simulink model "s_b8a4x128f"  (R2016b)
settings: Solver=VariableStepDiscrete  StartTime=0.0  StopTime=1  RelTol=1e-3
undefined symbols (not defined in the file): fft_stages, n_bits_ants, n_bits_xengs
libraries: xbsIndex_r4 x21069, casper_library_misc x164, casper_library_scopes x9, xbsReplacements_r4 x9, casper_library_delays x8, xps_library x3
(part 27 of 186)

== system s_b8a4x128f/sys1/bf_pack_out1 ==
  note: ensure sync_in
      | aligns with data
      | for storage
      | in FIFO
  note: rst turns off
      | as first data item
      | becomes available
      | at fifo
  note: insert dead time (based on clock rates and packet size) before transmission to guarantee this
      | packet will not overflow the fifo. Note that this assumes destination fifo at least as large as the packet
  note: if in reset report
      | end of file
      | immediately
  note: if there is an overflow, flush
      | all buffers and reset logic. Then
      | hold in reset till next sync
  note: increment heap offset
      | as packets leave
  note: keep space for
      | two timestamps/syncs
  note: change timestamp/sync
      | as last packet of
      | heap leaves
  note: capture timestamp on
      | first data item
      | of heap
  rst : Inport
  synci : Inport  Port=2
  di : Inport  Port=3
  eni : Inport  Port=4
  timei : Inport  Port=5
  start : Inport  Port=6
  id : Inport  Port=7
  Assert1 : xbsIndex_r4/Assert  assert_type=on  type_source=Explicitly  gui_display_data_type=Fixed-point  arith_type=Unsigned  n_bits=group_size_bits  bin_pt=0  preci_type=Single  exp_width=8  frac_width=24  assert_rate=off  rate_source=Explicitly  period=1  output_port=on  block_type=assert
      settings: block_version=11.4
  Assert{2,4,6,10} (4 alike) : xbsIndex_r4/Assert  assert_type=on  type_source=Explicitly  gui_display_data_type=Fixed-point  arith_type=Boolean  n_bits=1  bin_pt=0  preci_type=Single  exp_width=8  frac_width=24  assert_rate=off  rate_source=Explicitly  period=1  output_port=on  block_type=assert
      settings: block_version=11.4
  Assert5 : xbsIndex_r4/Assert  assert_type=on  type_source=Explicitly  gui_display_data_type=Fixed-point  arith_type=Unsigned  n_bits=spead_lsw  bin_pt=0  preci_type=Single  exp_width=8  frac_width=24  assert_rate=off  rate_source=Explicitly  period=1  output_port=on  block_type=assert
      settings: block_version=11.4
  Assert7 : xbsIndex_r4/Assert  assert_type=on  type_source=Explicitly  gui_display_data_type=Fixed-point  arith_type=Unsigned  n_bits=8*2^bit_width_in  bin_pt=0  preci_type=Single  exp_width=8  frac_width=24  assert_rate=off  rate_source=Explicitly  period=1  output_port=on  block_type=assert
      settings: block_version=11.4
  Concat{,1..3} (4 alike) : xbsIndex_r4/Concat  num_inputs=2  dbl_ovrd=off  block_type=concat
  Constant : xbsIndex_r4/Constant  const=0  gui_display_data_type=Fixed-point  arith_type=Signed (2's comp)  n_bits=heap_bits  bin_pt=0  preci_type=Single  exp_width=8  frac_width=24  explicit_period=off  period=1  equ=P=C  opselect=C  inp2=PCIN>>17  opr=+  inp1=P  carry=CIN  dbl_ovrd=off  block_type=constant
      settings: block_version=11.4
  Constant1 : xbsIndex_r4/Constant  const=0  gui_display_data_type=Fixed-point  arith_type=Unsigned  n_bits=48  bin_pt=0  preci_type=Single  exp_width=8  frac_width=24  explicit_period=on  period=1  equ=P=C  opselect=C  inp2=PCIN>>17  opr=+  inp1=P  carry=CIN  dbl_ovrd=off  block_type=constant
  Constant2 : xbsIndex_r4/Constant  const=2^(packet_bits-bit_width_out)  gui_display_data_type=Fixed-point  arith_type=Unsigned  n_bits=48  bin_pt=0  preci_type=Single  exp_width=8  frac_width=24  explicit_period=on  period=1  equ=P=C  opselect=C  inp2=PCIN>>17  opr=+  inp1=P  carry=CIN  dbl_ovrd=off  block_type=constant
  Constant3 : xbsIndex_r4/Constant  const=0  gui_display_data_type=Fixed-point  arith_type=Unsigned  n_bits=packet_bits  bin_pt=0  preci_type=Single  exp_width=8  frac_width=24  explicit_period=off  period=1  equ=P=C  opselect=C  inp2=PCIN>>17  opr=+  inp1=P  carry=CIN  dbl_ovrd=off  block_type=constant
      settings: block_version=11.4
  Constant5 : xbsIndex_r4/Constant  const=2^(heap_bits+bit_width_in)  gui_display_data_type=Fixed-point  arith_type=Unsigned  n_bits=48  bin_pt=0  preci_type=Single  exp_width=8  frac_width=24  explicit_period=on  period=1  equ=P=C  opselect=C  inp2=PCIN>>17  opr=+  inp1=P  carry=CIN  dbl_ovrd=off  block_type=constant
  Constant6 : xbsIndex_r4/Constant  const=0  gui_display_data_type=Fixed-point  arith_type=Unsigned  n_bits=n_bits_chans  bin_pt=0  preci_type=Single  exp_width=8  frac_width=24  explicit_period=off  period=1  equ=P=C  opselect=C  inp2=PCIN>>17  opr=+  inp1=P  carry=CIN  dbl_ovrd=off  block_type=constant
      settings: block_version=11.4
  Convert : xbsIndex_r4/Convert  gui_display_data_type=Fixed-point  arith_type=Unsigned  n_bits=spead_lsw  bin_pt=0  float_type=Single  exp_bits=8  fraction_bits=24  quantization=Truncate  overflow=Wrap  en=off  latency=0  pipeline=off  dbl_ovrd=off  block_type=convert
  Convert1 : xbsIndex_r4/Convert  gui_display_data_type=Fixed-point  arith_type=Unsigned  n_bits=spead_lsw  bin_pt=0  float_type=Single  exp_bits=8  fraction_bits=24  quantization=Truncate  overflow=Wrap  en=off  latency=0  pipeline=off  dbl_ovrd=off  block_type=convert
  Convert2 : xbsIndex_r4/Convert  gui_display_data_type=Fixed-point  arith_type=Unsigned  n_bits=spead_lsw  bin_pt=0  float_type=Single  exp_bits=8  fraction_bits=24  quantization=Truncate  overflow=Wrap  en=off  latency=0  pipeline=off  dbl_ovrd=off  block_type=convert
  Delay{,1..11,17,19..20} (15 alike) : xbsIndex_r4/Delay  rst=off  infoeditControl=Selection of Reset will increase slice count due to use of real FFs and instead of SRLs  en=off  latency=1  reg_retiming=on  dbl_ovrd=off  block_type=delay
      settings: block_version=11.4
  Delay12 : xbsIndex_r4/Delay  rst=off  infoeditControl=Selection of Reset will increase slice count due to use of real FFs and instead of SRLs  en=off  latency=0  reg_retiming=on  dbl_ovrd=off  block_type=delay
      settings: block_version=11.4
  Gateway Out{,1..16} (17 alike) : xbsIndex_r4/Gateway Out  inherit_from_input=off  hdl_port=off  rows=1  columns=1  UseAsDAC=off  DACChannel='1'  interface=None  automatic_assignment=on  address_offset=hex2dec('00')  intf_name=''  intf_description=''  timing_constraint=None  locs_specified=off  LOCs={}  io_standard={}  block_type=gatewayout
      settings: infoedit="Gateway out block.  Converts Xilinx fixed point inputs into ouputs of type Simulink integer, double, or fixed point.<br><br>Hardware notes:  In hardware these blocks become top level output ports or are discarded, depending on how they are configured."  block_version=11.4
  Inverter{,1..5} (6 alike) : xbsIndex_r4/Inverter  en=off  latency=0  dbl_ovrd=off  block_type=inv
      Inverter1 settings: block_version=11.4
      Inverter2 settings: block_version=11.4
      Inverter3 settings: block_version=11.4
      Inverter4 settings: block_version=11.4
  Logical : xbsIndex_r4/Logical  logical_function=AND  inputs=2  en=off  latency=1  precision=Full  arith_type=Unsigned  n_bits=16  bin_pt=0  align_bp=on  dbl_ovrd=off  block_type=logical
      settings: block_version=11.4
  Logical{1,3..4,6} (4 alike) : xbsIndex_r4/Logical  logical_function=AND  inputs=2  en=off  latency=0  precision=Full  arith_type=Unsigned  n_bits=16  bin_pt=0  align_bp=on  dbl_ovrd=off  block_type=logical
      settings: block_version=11.4
  Logical10 : xbsIndex_r4/Logical  logical_function=OR  inputs=2  en=off  latency=0  precision=Full  arith_type=Unsigned  n_bits=16  bin_pt=0  align_bp=on  dbl_ovrd=off  block_type=logical
      settings: block_version=11.4
  Logical2 : xbsIndex_r4/Logical  logical_function=AND  inputs=3  en=off  latency=1  precision=Full  arith_type=Unsigned  n_bits=16  bin_pt=0  align_bp=on  dbl_ovrd=off  block_type=logical
      settings: block_version=11.4
  Logical5 : xbsIndex_r4/Logical  logical_function=OR  inputs=2  en=off  latency=1  precision=Full  arith_type=Unsigned  n_bits=16  bin_pt=0  align_bp=on  dbl_ovrd=off  block_type=logical
      settings: block_version=11.4
  Logical8 : xbsIndex_r4/Logical  logical_function=OR  inputs=2  en=off  latency=0  precision=Full  arith_type=Unsigned  n_bits=16  bin_pt=0  align_bp=on  dbl_ovrd=off  block_type=logical
      settings: block_version=11.4
  Logical9 : xbsIndex_r4/Logical  logical_function=OR  inputs=2  en=off  latency=0  precision=Full  arith_type=Unsigned  n_bits=16  bin_pt=0  align_bp=on  dbl_ovrd=off  block_type=logical
  Register : xbsIndex_r4/Register  init=0  rst=on  en=on  dbl_ovrd=off  block_type=register
      settings: block_version=11.4
  Register2 : xbsIndex_r4/Register  init=0  rst=on  en=on  dbl_ovrd=off  block_type=register
  Reinterpret : xbsIndex_r4/Reinterpret  force_arith_type=on  arith_type="Signed  (2's comp)"  force_bin_pt=on  bin_pt=0  block_type=reinterpret
      settings: infoedit="Changes signal type without altering the binary representation.   You can changed the signal between signed and unsigned, and relocate the binary point.<br><br>Hardware notes: In hardware this block costs nothing.<br><br>Example:  Suppose the input is 6 bits wide, signed, with 2 fractional bits, and the output is forced to unsigned with 0 fractional bits.  Then an input of -2.0 (1110.00 in binary 2's complement) becomes an output of 56 (111000 in binary)."
  Reinterpret1 : xbsIndex_r4/Reinterpret  force_arith_type=on  arith_type="Signed  (2's comp)"  force_bin_pt=on  bin_pt=0  block_type=reinterpret
      settings: infoedit="Changes signal type without altering the binary representation.   You can changed the signal between signed and unsigned, and relocate the binary point.<br><br>Hardware notes: In hardware this block costs nothing.<br><br>Example:  Suppose the input is 6 bits wide, signed, with 2 fractional bits, and the output is forced to unsigned with 0 fractional bits.  Then an input of -2.0 (1110.00 in binary 2's complement) becomes an output of 56 (111000 in binary)."
  Reinterpret2 : xbsIndex_r4/Reinterpret  force_arith_type=on  arith_type="Signed  (2's comp)"  force_bin_pt=on  bin_pt=0  block_type=reinterpret
      settings: infoedit="Changes signal type without altering the binary representation.   You can changed the signal between signed and unsigned, and relocate the binary point.<br><br>Hardware notes: In hardware this block costs nothing.<br><br>Example:  Suppose the input is 6 bits wide, signed, with 2 fractional bits, and the output is forced to unsigned with 0 fractional bits.  Then an input of -2.0 (1110.00 in binary 2's complement) becomes an output of 56 (111000 in binary)."
  Relational : xbsIndex_r4/Relational  mode=a=b  op_type=Bool  en=off  latency=0  dbl_ovrd=off  block_type=relational
  Relational1 : xbsIndex_r4/Relational  mode=a<b  op_type=Bool  en=off  latency=1  dbl_ovrd=off  block_type=relational
  Scope : Scope  NumInputPorts=8
  Scope1 : Scope  NumInputPorts=7
  Scope2 : Scope  NumInputPorts=2
  Slice2 : xbsIndex_r4/Slice  nbits=2^bit_width_in*8/2  boolean_output=off  mode=Upper Bit Location + Width  bit1=0  base1=MSB of Input  bit0=0  base0=LSB of Input  dbl_ovrd=off  block_type=slice
  Slice3 : xbsIndex_r4/Slice  nbits=2^bit_width_in*8/2  boolean_output=off  mode=Lower Bit Location + Width  bit1=0  base1=LSB of Input  bit0=0  base0=LSB of Input  dbl_ovrd=off  block_type=slice
  Slice4 : xbsIndex_r4/Slice  nbits=1  boolean_output=on  mode=Upper Bit Location + Width  bit1=0  base1=MSB of Input  bit0=0  base0=LSB of Input  dbl_ovrd=off  block_type=slice
  Slice5 : xbsIndex_r4/Slice  nbits=2^bit_width_in*8/4  boolean_output=off  mode=Upper Bit Location + Width  bit1=0  base1=MSB of Input  bit0=0  base0=LSB of Input  dbl_ovrd=off  block_type=slice
  Slice7 : xbsIndex_r4/Slice  nbits=1  boolean_output=on  mode=Upper Bit Location + Width  bit1=0  base1=MSB of Input  bit0=0  base0=LSB of Input  dbl_ovrd=off  block_type=slice
  Slice8 : xbsIndex_r4/Slice  nbits=spead_lsw  boolean_output=off  mode=Lower Bit Location + Width  bit1=0  base1=MSB of Input  bit0=0  base0=LSB of Input  dbl_ovrd=off  block_type=slice
  Subsystem3 : Subsystem
  conv : xbsIndex_r4/Slice  nbits=1  boolean_output=on  mode=Upper Bit Location + Width  bit1=0  base1=MSB of Input  bit0=0  base0=LSB of Input  dbl_ovrd=off  block_type=slice
  count_in : xbsIndex_r4/Counter  cnt_type=Free Running  cnt_to=Inf  operation=Up  start_count=0  cnt_by_val=1  arith_type=Unsigned  n_bits=heap_bits  bin_pt=0  load_pin=off  rst=on  en=on  explicit_period=on  period=1  use_behavioral_HDL=on  implementation=Fabric  dbl_ovrd=off  block_type=counter
      settings: block_version=11.4
  data_fifo : Subsystem  mask{depth_bits=log2(2*(8*2^packet_bits)/(8*2^bit_width_in)), scale_bits=bit_width_out-bit_width_in, full_bits=1, n_bits_in=8*2^bit_width_in}
      mask prompts: depth_bits "depth (2^?)"; scale_bits "output data width scale factor (2^?)"; full_bits "number of bits for %full signal"; n_bits_in "word size"
      mask init: same as s_b8a4x128f/sys0/bf_pack_out0/data_fifo
  dead_count : xbsIndex_r4/Counter  cnt_type=Free Running  cnt_to=Inf  operation=Up  start_count=0  cnt_by_val=1  arith_type=Unsigned  n_bits=ceil(log2(ceil(((fabric_clock-tx_clock)/tx_clock)*(2^(packet_bits-3)+7))))  bin_pt=0  load_pin=off  rst=on  en=on  explicit_period=on  period=1  use_behavioral_HDL=on  implementation=Fabric  dbl_ovrd=off  block_type=counter
      settings: block_version=11.4
  edge_detect : Subsystem  AncestorBlock=casper_library_misc/edge_detect  mask(edge_detect){edge=Rising, polarity=Active High, x_in=[0 0.08 0.08 0.16 0.16 0.24 0.24 0.32 0.32 0.4], y_in=[-1 -1  1  1  1  1  1  1  1  1], x_out=[0.6 0.68 0.68 0.76 0.76 0.84 0.84 0.92 0.92 1], y_out=[-1 -1  1  1 -1 -1 -1 -1 -1 -1]}
      mask prompts: edge "Edge Type"; polarity "Output Polarity"; x_in "Input X Positions"; y_in "Input Y Positions"; x_out "Output X Positions"; y_out "Output Y Positions"
      mask help: Output is active for one-cycle after each edge of the specified type (i.e. rising, falling or both).
      mask init: same as s_b8a4x128f/edge_detect
      settings: AttributesFormatString=|
      | rising edges
      | active high
      mask Help: Output is active for one-cycle after each edge of the specified type (i.e. rising, falling, or both).  Latency is zero.
      mask TypeOptions edge: Rising | Falling | Both
      mask TypeOptions polarity: Active High | Active Low
      mask Display:
      | plot(x_in_num,0.5+y_in_num*0.2);
      | plot(x_out_num,0.5+y_out_num*0.2);
  edge_detect2 : Subsystem  AncestorBlock=casper_library_misc/edge_detect  mask(edge_detect){edge=Rising, polarity=Active High, x_in=[0 0.08 0.08 0.16 0.16 0.24 0.24 0.32 0.32 0.4], y_in=[-1 -1  1  1  1  1  1  1  1  1], x_out=[0.6 0.68 0.68 0.76 0.76 0.84 0.84 0.92 0.92 1], y_out=[-1 -1  1  1 -1 -1 -1 -1 -1 -1]}
      mask prompts: edge "Edge Type"; polarity "Output Polarity"; x_in "Input X Positions"; y_in "Input Y Positions"; x_out "Output X Positions"; y_out "Output Y Positions"
      mask help: Output is active for one-cycle after each edge of the specified type (i.e. rising, falling or both).
      mask init: same as s_b8a4x128f/edge_detect
      settings: AttributesFormatString=|
      | rising edges
      | active high
      mask Help: Output is active for one-cycle after each edge of the specified type (i.e. rising, falling, or both).  Latency is zero.
      mask TypeOptions edge: Rising | Falling | Both
      mask TypeOptions polarity: Active High | Active Low
      mask Display:
      | plot(x_in_num,0.5+y_in_num*0.2);
      | plot(x_out_num,0.5+y_out_num*0.2);
  edge_detect3 : Subsystem  AncestorBlock=casper_library_misc/edge_detect  mask(edge_detect){edge=Rising, polarity=Active High, x_in=[0 0.08 0.08 0.16 0.16 0.24 0.24 0.32 0.32 0.4], y_in=[-1 -1  1  1  1  1  1  1  1  1], x_out=[0.6 0.68 0.68 0.76 0.76 0.84 0.84 0.92 0.92 1], y_out=[-1 -1  1  1 -1 -1 -1 -1 -1 -1]}
      mask prompts: edge "Edge Type"; polarity "Output Polarity"; x_in "Input X Positions"; y_in "Input Y Positions"; x_out "Output X Positions"; y_out "Output Y Positions"
      mask help: Output is active for one-cycle after each edge of the specified type (i.e. rising, falling or both).
      mask init: same as s_b8a4x128f/edge_detect
      settings: AttributesFormatString=|
      | rising edges
      | active high
      mask Help: Output is active for one-cycle after each edge of the specified type (i.e. rising, falling, or both).  Latency is zero.
      mask TypeOptions edge: Rising | Falling | Both
      mask TypeOptions polarity: Active High | Active Low
      mask Display:
      | plot(x_in_num,0.5+y_in_num*0.2);
      | plot(x_out_num,0.5+y_out_num*0.2);
  edge_detect4 : Subsystem  AncestorBlock=casper_library_misc/edge_detect  mask(edge_detect){edge=Rising, polarity=Active High, x_in=[0 0.08 0.08 0.16 0.16 0.24 0.24 0.32 0.32 0.4], y_in=[-1 -1  1  1  1  1  1  1  1  1], x_out=[0.6 0.68 0.68 0.76 0.76 0.84 0.84 0.92 0.92 1], y_out=[-1 -1  1  1 -1 -1 -1 -1 -1 -1]}
      mask prompts: edge "Edge Type"; polarity "Output Polarity"; x_in "Input X Positions"; y_in "Input Y Positions"; x_out "Output X Positions"; y_out "Output Y Positions"
      mask help: Output is active for one-cycle after each edge of the specified type (i.e. rising, falling or both).
      mask init: same as s_b8a4x128f/edge_detect
      settings: AttributesFormatString=|
      | rising edges
      | active high
      mask Help: Output is active for one-cycle after each edge of the specified type (i.e. rising, falling, or both).  Latency is zero.
      mask TypeOptions edge: Rising | Falling | Both
      mask TypeOptions polarity: Active High | Active Low
      mask Display:
      | plot(x_in_num,0.5+y_in_num*0.2);
      | plot(x_out_num,0.5+y_out_num*0.2);
  edge_detect7 : Subsystem  AncestorBlock=casper_library_misc/edge_detect  mask(edge_detect){edge=Rising, polarity=Active High, x_in=[0 0.08 0.08 0.16 0.16 0.24 0.24 0.32 0.32 0.4], y_in=[-1 -1  1  1  1  1  1  1  1  1], x_out=[0.6 0.68 0.68 0.76 0.76 0.84 0.84 0.92 0.92 1], y_out=[-1 -1  1  1 -1 -1 -1 -1 -1 -1]}
      mask prompts: edge "Edge Type"; polarity "Output Polarity"; x_in "Input X Positions"; y_in "Input Y Positions"; x_out "Output X Positions"; y_out "Output Y Positions"
      mask help: Output is active for one-cycle after each edge of the specified type (i.e. rising, falling or both).
      mask init: same as s_b8a4x128f/edge_detect
      settings: AttributesFormatString=|
      | rising edges
      | active high
      mask Help: Output is active for one-cycle after each edge of the specified type (i.e. rising, falling, or both).  Latency is zero.
      mask TypeOptions edge: Rising | Falling | Both
      mask TypeOptions polarity: Active High | Active Low
      mask Display:
      | plot(x_in_num,0.5+y_in_num*0.2);
      | plot(x_out_num,0.5+y_out_num*0.2);
  gap_size : xbsIndex_r4/Constant  const=ceil(((fabric_clock-tx_clock)/tx_clock)*(2^(packet_bits-3)+7))  gui_display_data_type=Fixed-point  arith_type=Unsigned  n_bits=ceil(log2(ceil(((fabric_clock-tx_clock)/tx_clock)*(2^(packet_bits-3)+7))))  bin_pt=0  preci_type=Single  exp_width=8  frac_width=24  explicit_period=on  period=1  equ=P=C  opselect=C  inp2=PCIN>>17  opr=+  inp1=P  carry=CIN  dbl_ovrd=off  block_type=constant
      settings: block_version=11.4
  in_dest : xbsIndex_r4/Counter  cnt_type=Free Running  cnt_to=Inf  operation=Up  start_count=0  cnt_by_val=1  arith_type=Unsigned  n_bits=1  bin_pt=0  load_pin=off  rst=on  en=on  explicit_period=on  period=1  use_behavioral_HDL=on  implementation=Fabric  dbl_ovrd=off  block_type=counter
      settings: block_version=11.4
  msb : xbsIndex_r4/Slice  nbits=1  boolean_output=on  mode=Upper Bit Location + Width  bit1=0  base1=MSB of Input  bit0=0  base0=LSB of Input  dbl_ovrd=off  block_type=slice
  mux : xbsIndex_r4/Mux  inputs=2  en=off  latency=1  precision=Full  arith_type=Unsigned  n_bits=16  bin_pt=14  quantization=Truncate  overflow=Wrap  dbl_ovrd=off  block_type=mux
      settings: block_version=11.4
  offset_cnt : xbsIndex_r4/Counter  cnt_type=Free Running  cnt_to=Inf  operation=Up  start_count=0  cnt_by_val=1  arith_type=Unsigned  n_bits=(heap_bits+bit_width_in)-packet_bits  bin_pt=0  load_pin=off  rst=on  en=on  explicit_period=on  period=1  use_behavioral_HDL=on  implementation=Fabric  dbl_ovrd=off  block_type=counter
      settings: block_version=11.4
  out_src : xbsIndex_r4/Counter  cnt_type=Free Running  cnt_to=Inf  operation=Up  start_count=0  cnt_by_val=1  arith_type=Unsigned  n_bits=(heap_bits+bit_width_in)-packet_bits+1  bin_pt=0  load_pin=off  rst=on  en=on  explicit_period=on  period=1  use_behavioral_HDL=on  implementation=Fabric  dbl_ovrd=off  block_type=counter
      settings: block_version=11.4
  pack : Subsystem  mask(pkt_pack_mask){pkt_bits=packet_bits-bit_width_out, fifo_latency=4, spead_msw=spead_msw, spead_lsw=spead_lsw}
      mask prompts: pkt_bits "Payload Length (2^?)"; fifo_latency "Fifo latency"; spead_msw "SPEAD Flavour (MSw)"; spead_lsw "SPEAD Flavour (LSw)"
      mask help:
      | This block generates SPEAD-compliant packets from a datastream.
      |
      | Packets are created with a fixed header followed by a number of 64-bit items.
      |
      | Requires a 64-bit data stream.
      |
      | See the documentation for further details.
  spead_pack : Subsystem  Tag=casper:spead_pack  AncestorBlock=casper_library_communications/spead_pack  mask(pkt_pack_mask){max_pkt_len_bits=9, header_ids=0x1600, 0x4103, header_ind_ids=0x4300, spead_msw=64, spead_lsw=48, spead_version=4, bytes_per_word=8}
      mask prompts: max_pkt_len_bits "Max pkt length, 2^? 64-bit words"; header_ids "SPEAD direct address IDs (decimal)"; header_ind_ids "SPEAD indirect address IDs (decimal)"; spead_msw "SPEAD Flavour (MSw)"; spead_lsw "SPEAD Flavour (LSw)"; spead_version "SPEAD version"; bytes_per_word "Word size, in bytes"
      mask help:
      | This block generates SPEAD-compliant packets from a datastream.
      |
      | Packets are created with a fixed header followed by a number of 64-bit items.
      |
      | Requires a 64-bit data stream.
      |
      | The data_ready signal is one cycle BEFORE valid data! Does not have to be with a valid signal either.
      mask init:
      | % if floor(log2(bytes_per_word)) ~= log2(bytes_per_word)
      | %     error('Bytes per word should be a power of two.');
      | % end
      | % 
      | % spead_pack_init(gcb)
  status : Subsystem  Tag=xps:sw_reg  AncestorBlock=xps_library/software register  mask(swreg){io_dir=To Processor, io_delay=0, sample_period=1, names=[pkt_cnt fifo_of_err_cnt], bitwidths=16, bin_pts=0, arith_types=0, sim_port=off, show_format=on}
      mask prompts: io_dir "I/O direction"; io_delay "I/O delay"; sample_period "Sample period"; names "Bitfield names [msb...lsb]"; bitwidths "Bitfield widths"; bin_pts "Bitfield binary pts"; arith_types "Bitfield types, ufix=0, fix=1, bool=2"; sim_port "Provide sim input/output?"; show_format "Print format string?"
      mask help: A 32-bit software-accessible register. Can be divided into bitfields of varying widths and types using the fields in the block mask.
      mask init:
      | try
      |     swreg_init(gcb)
      | catch ex
      |     disp(sprintf('%s: %s', gcb, ex.message))
      |     errordlg(ex.message)
      | end
      settings: AttributesFormatString=2 outputs:uf16.0,uf16.0 = 32 bits
      mask TypeOptions io_dir: To Processor | From Processor
      mask Callback io_dir:
      | mask_enables = get_param(gcb, 'MaskEnables');
      | mask_names = get_param(gcb, 'MaskNames');
      | if strcmp(get_param(gcb, 'io_dir'), 'To Processor'),
      |     mask_enables{ismember(mask_names, 'sample_period')} = 'off';
      | else
      |     mask_enables{ismember(mask_names, 'sample_period')} = 'on';
      | end
      | set_param(gcb, 'MaskEnables', mask_enables);
  time0 : xbsIndex_r4/Register  init=0  rst=off  en=on  dbl_ovrd=off  block_type=register
      settings: block_version=11.4
  time1 : xbsIndex_r4/Register  init=0  rst=off  en=on  dbl_ovrd=off  block_type=register
      settings: block_version=11.4
  do : Outport
  eno : Outport  Port=2
  eofo : Outport  Port=3
  pkt_ready : Outport  Port=4
  wires:
  [id] -> Concat3/2
  [time_out] -> Concat3/1
  Convert2/1 -> spead_pack/6(hdr_heap_offset), Gateway Out3/1
  Convert1/1 -> spead_pack/4(hdr_heap_id)
  Concat3/1 -> Convert1/1
  [id] -> Concat2/1
  Convert/1 -> spead_pack/9(hdr6_0x4103_DIR)
  Constant6/1 -> Concat2/2
  Concat2/1 -> Convert/1
  Constant5/1 -> spead_pack/5(hdr_heap_size)
  Constant2/1 -> spead_pack/7(hdr_pkt_len_words)
  [time_out] -> spead_pack/8(hdr5_0x1600_DIR)
  Constant1/1 -> spead_pack/10(hdr8_0x5000)
  Delay9/1 -> Delay7/1
  spead_pack/2(valid_out) -> Delay11/1
  spead_pack/1(data_out) -> Delay10/1
  Delay8/1 -> spead_pack/1(data256_ready)
  Delay7/1 -> Delay8/1
  Delay4/1 -> Delay9/1
  Delay6/1 -> spead_pack/2(data256_valid)
  Delay5/1 -> Delay6/1
  pack/1(pkt_start) -> Delay4/1
  Delay3/1 -> spead_pack/3(data256), Slice2/1, Slice3/1
  spead_pack/3(eof) -> Logical5/2, [eof]
  Logical10/1 -> offset_cnt/1
  [rst_fifo] -> Logical10/2
  [sync_out] -> Logical10/1
  msb/1 -> mux/1
  edge_detect2/1(out) -> Register/3, Register/1
  Logical9/1 -> Register/2
  Inverter5/1 -> Delay12/1
  [of] -> Logical9/2
  [rst_in] -> Logical9/1
  Assert10/1 -> [rst_in]
  rst/1 -> Assert10/1
  [time_we] -> Register2/1, Register2/3
  edge_detect7/1(out) -> [sync_out]
  edge_detect4/1(out) -> Register2/2
  Inverter/1 -> Concat1/1
  [sync_in] -> edge_detect4/1(in)
  [sync_in] -> Gateway Out15/1
  Slice8/1 -> [time_out]
  Slice7/1 -> edge_detect7/1(in)
  mux/1 -> Slice8/1, Slice7/1
  Concat1/1 -> Gateway Out10/1, time0/1, time1/1
  Delay/1 -> Concat1/2
  Register2/1 -> Inverter/1
  [rst_fifo] -> Logical6/2
  Logical8/1 -> Logical6/1
  [start_ext] -> Logical8/2
  [start] -> Logical8/1
  Logical1/1 -> dead_count/1
  edge_detect3/1(out) -> Logical1/2
  Inverter4/1 -> Logical1/1
  [rst_fifo] -> Inverter4/1
  [sync_out] -> Gateway Out13/1
  [rst_fifo] -> out_src/1
  [eof] -> out_src/2
  [rst_fifo] -> in_dest/1
  Gateway Out15/1 -> Scope1/7
  Delay20/1 -> Gateway Out8/1
  Delay12/1 -> [rst_fifo]
  data_fifo/1(do) -> Delay3/1
  Delay19/1 -> Slice5/1, data_fifo/3(di)
  Assert7/1 -> Delay19/1
  Assert6/1 -> Delay17/1
  Assert5/1 -> Delay/1
  Assert4/1 -> [sync_in]
  Gateway Out16/1 -> Scope2/2
  Gateway Out14/1 -> Scope2/1
  di/1 -> Assert7/1
  Inverter3/1 -> Logical2/3
  [rst_fifo] -> Inverter3/1
  Inverter2/1 -> edge_detect/1(in)
  Relational1/1 -> Inverter2/1, dead_count/2
  Assert2/1 -> edge_detect3/1(in), [start_ext]
  gap_size/1 -> Relational1/2
  dead_count/1 -> Relational1/1
  start/1 -> Assert2/1
  Logical6/1 -> Logical5/1
  Logical5/1 -> eofo/1
  Delay17/1 -> Gateway Out7/1, data_fifo/2(we)
  [start] -> Logical2/2
  edge_detect/1(out) -> [start]
  [rst_fifo] -> Gateway Out16/1
  [of] -> Gateway Out14/1
  [sync_in] -> edge_detect2/1(in)
  Assert1/1 -> Gateway Out2/1, [id]
  Constant/1 -> Relational/2
  Relational/1 -> Logical/1
  Register/1 -> Inverter5/1
  synci/1 -> Assert4/1
  data_fifo/3(of) -> [of]
  Inverter1/1 -> Logical3/2
  [time_out] -> Gateway Out4/1
  time1/1 -> mux/3
  time0/1 -> mux/2
  out_src/1 -> msb/1
  Logical4/1 -> time1/2
  conv/1 -> Inverter1/1, Logical4/2
  Logical3/1 -> time0/2
  in_dest/1 -> conv/1
  [eof] -> offset_cnt/2
  [pkt_ready] -> Logical2/1
  Gateway Out13/1 -> Scope/8
  Reinterpret2/1 -> Gateway Out6/1
  Slice5/1 -> Reinterpret2/1
  Reinterpret1/1 -> Gateway Out12/1
  Reinterpret/1 -> Gateway Out5/1
  Constant3/1 -> Concat/2
  offset_cnt/1 -> Gateway Out1/1, Gateway Out/1, [offset_cnt], Concat/1
  id/1 -> Assert1/1
  Slice4/1 -> [pkt_ready], pkt_ready/1
  Slice3/1 -> Reinterpret1/1
  Gateway Out12/1 -> Scope/7
  Slice2/1 -> Reinterpret/1
  Gateway Out11/1 -> Scope1/6
  Gateway Out10/1 -> Scope1/5
  Gateway Out9/1 -> Scope1/4
  Gateway Out8/1 -> Scope1/3
  Gateway Out7/1 -> Scope1/2
  Gateway Out6/1 -> Scope1/1
  [pkt_ready] -> Gateway Out11/1
  Gateway Out5/1 -> Scope/6
  Gateway Out4/1 -> Scope/5
  Gateway Out3/1 -> Scope/4
  Gateway Out2/1 -> Scope/3
  Gateway Out1/1 -> Scope/2
  Gateway Out/1 -> Scope/1
  Concat/1 -> Convert2/1
  data_fifo/2(%full) -> Slice4/1
  [sync_in] -> count_in/1
  Logical/1 -> in_dest/2, Logical3/1, Gateway Out9/1, [time_we], Logical4/1
  count_in/1 -> Delay20/1, Relational/1
  Delay2/1 -> Delay5/1, data_fifo/4(re)
  timei/1 -> Assert5/1
  eni/1 -> count_in/2, Logical/2, Assert6/1
  [rst_fifo] -> data_fifo/1(rst)
  Delay1/1 -> Delay2/1
  pack/2(ack_out) -> Delay1/1
  Delay10/1 -> do/1
  Logical2/1 -> pack/1(pkt_rdy)
  Delay11/1 -> eno/1
  Subsystem3/1(Out1) -> status/1(out_pkt_cnt)
  [cnt_rst] -> Subsystem3/1(rst)
  [eof] -> Subsystem3/2(in0)
  [of] -> Subsystem3/3(in1)
  Subsystem3/2(Out2) -> status/2(out_fifo_of_err_cnt)

== system s_b8a4x128f/sys1/pipeline ==
  d : Inport
  Register0 : xbsIndex_r4/Register  init=0  rst=off  en=off  dbl_ovrd=off  block_type=register
      settings: block_version=11.4
  Register1 : xbsIndex_r4/Register  init=0  rst=off  en=off  dbl_ovrd=off  block_type=register
      settings: block_version=11.4
  q : Outport
  wires:
  Register1/1 -> q/1
  d/1 -> Register0/1
  Register0/1 -> Register1/1

== system s_b8a4x128f/sys1/pipeline1 ==
  d : Inport
  Register0 : xbsIndex_r4/Register  init=0  rst=off  en=off  dbl_ovrd=off  block_type=register
      settings: block_version=11.4
  Register1 : xbsIndex_r4/Register  init=0  rst=off  en=off  dbl_ovrd=off  block_type=register
      settings: block_version=11.4
  q : Outport
  wires:
  Register0/1 -> Register1/1
  d/1 -> Register0/1
  Register1/1 -> q/1

== system s_b8a4x128f/sys1/pipeline10 ==
  d : Inport
  Register0 : xbsIndex_r4/Register  init=0  rst=off  en=off  dbl_ovrd=off  block_type=register
      settings: block_version=11.4
  Register1 : xbsIndex_r4/Register  init=0  rst=off  en=off  dbl_ovrd=off  block_type=register
      settings: block_version=11.4
  q : Outport
  wires:
  Register1/1 -> q/1
  d/1 -> Register0/1
  Register0/1 -> Register1/1

== system s_b8a4x128f/sys1/pipeline11 ==
  d : Inport
  Register0 : xbsIndex_r4/Register  init=0  rst=off  en=off  dbl_ovrd=off  block_type=register
      settings: block_version=11.4
  Register1 : xbsIndex_r4/Register  init=0  rst=off  en=off  dbl_ovrd=off  block_type=register
      settings: block_version=11.4
  q : Outport
  wires:
  Register1/1 -> q/1
  d/1 -> Register0/1
  Register0/1 -> Register1/1

== system s_b8a4x128f/sys1/pipeline12 ==
  d : Inport
  Register0 : xbsIndex_r4/Register  init=0  rst=off  en=off  dbl_ovrd=off  block_type=register
      settings: block_version=11.4
  Register1 : xbsIndex_r4/Register  init=0  rst=off  en=off  dbl_ovrd=off  block_type=register
      settings: block_version=11.4
  q : Outport
  wires:
  Register0/1 -> Register1/1
  d/1 -> Register0/1
  Register1/1 -> q/1

== system s_b8a4x128f/sys1/pipeline13 ==
  d : Inport
  Register0 : xbsIndex_r4/Register  init=0  rst=off  en=off  dbl_ovrd=off  block_type=register
      settings: block_version=11.4
  Register1 : xbsIndex_r4/Register  init=0  rst=off  en=off  dbl_ovrd=off  block_type=register
      settings: block_version=11.4
  q : Outport
  wires:
  Register1/1 -> q/1
  d/1 -> Register0/1
  Register0/1 -> Register1/1

== system s_b8a4x128f/sys1/pipeline2 ==
  d : Inport
  Register0 : xbsIndex_r4/Register  init=0  rst=off  en=off  dbl_ovrd=off  block_type=register
      settings: block_version=11.4
  Register1 : xbsIndex_r4/Register  init=0  rst=off  en=off  dbl_ovrd=off  block_type=register
      settings: block_version=11.4
  q : Outport
  wires:
  Register1/1 -> q/1
  d/1 -> Register0/1
  Register0/1 -> Register1/1

== system s_b8a4x128f/sys1/pipeline3 ==
  d : Inport
  Register0 : xbsIndex_r4/Register  init=0  rst=off  en=off  dbl_ovrd=off  block_type=register
      settings: block_version=11.4
  Register1 : xbsIndex_r4/Register  init=0  rst=off  en=off  dbl_ovrd=off  block_type=register
      settings: block_version=11.4
  q : Outport
  wires:
  Register0/1 -> Register1/1
  d/1 -> Register0/1
  Register1/1 -> q/1

== system s_b8a4x128f/sys1/pipeline4 ==
  d : Inport
  Register0 : xbsIndex_r4/Register  init=0  rst=off  en=off  dbl_ovrd=off  block_type=register
      settings: block_version=11.4
  Register1 : xbsIndex_r4/Register  init=0  rst=off  en=off  dbl_ovrd=off  block_type=register
      settings: block_version=11.4
  q : Outport
  wires:
  Register1/1 -> q/1
  d/1 -> Register0/1
  Register0/1 -> Register1/1

== system s_b8a4x128f/sys1/pipeline5 ==
  d : Inport
  Register0 : xbsIndex_r4/Register  init=0  rst=off  en=off  dbl_ovrd=off  block_type=register
      settings: block_version=11.4
  Register1 : xbsIndex_r4/Register  init=0  rst=off  en=off  dbl_ovrd=off  block_type=register
      settings: block_version=11.4
  q : Outport
  wires:
  Register1/1 -> q/1
  d/1 -> Register0/1
  Register0/1 -> Register1/1

== system s_b8a4x128f/sys1/pipeline6 ==
  d : Inport
  Register0 : xbsIndex_r4/Register  init=0  rst=off  en=off  dbl_ovrd=off  block_type=register
      settings: block_version=11.4
  Register1 : xbsIndex_r4/Register  init=0  rst=off  en=off  dbl_ovrd=off  block_type=register
      settings: block_version=11.4
  q : Outport
  wires:
  Register0/1 -> Register1/1
  d/1 -> Register0/1
  Register1/1 -> q/1

== system s_b8a4x128f/sys1/pipeline7 ==
  d : Inport
  Register0 : xbsIndex_r4/Register  init=0  rst=off  en=off  dbl_ovrd=off  block_type=register
      settings: block_version=11.4
  Register1 : xbsIndex_r4/Register  init=0  rst=off  en=off  dbl_ovrd=off  block_type=register
      settings: block_version=11.4
  q : Outport
  wires:
  Register1/1 -> q/1
  d/1 -> Register0/1
  Register0/1 -> Register1/1

== system s_b8a4x128f/sys1/pipeline8 ==
  d : Inport
  Register0 : xbsIndex_r4/Register  init=0  rst=off  en=off  dbl_ovrd=off  block_type=register
      settings: block_version=11.4
  Register1 : xbsIndex_r4/Register  init=0  rst=off  en=off  dbl_ovrd=off  block_type=register
      settings: block_version=11.4
  q : Outport
  wires:
  Register0/1 -> Register1/1
  d/1 -> Register0/1
  Register1/1 -> q/1

== system s_b8a4x128f/sys1/pipeline9 ==
  d : Inport
  Register0 : xbsIndex_r4/Register  init=0  rst=off  en=off  dbl_ovrd=off  block_type=register
      settings: block_version=11.4
  Register1 : xbsIndex_r4/Register  init=0  rst=off  en=off  dbl_ovrd=off  block_type=register
      settings: block_version=11.4
  q : Outport
  wires:
  Register0/1 -> Register1/1
  d/1 -> Register0/1
  Register1/1 -> q/1
